simulink model "TB05_StageC_CLLC"  (R2025a)
settings: Solver=FixedStepDiscrete  StartTime=0  StopTime=TB.t_end  FixedStep=TB.dt  RelTol=1e-3
InitFcn:
  | % 모델과 같은 폴더의 초기화 스크립트를 실행해 P(설계 파라미터)와 TB(시험 조건)를 만든다.
  | run(fullfile(fileparts(get_param(bdroot, 'FileName')), 'TB05_init.m'));
values from neighbouring files (symbols this model uses):
  TB = struct()    [TB05_init.m]    (also in probe_TB05_solver.m = evalin('base', 'TB'); run_TB05.m = evalin('base', 'TB'))
libraries: fl_lib x35, nesl_utility x13
settings Model: Creator=hj000  LastModifiedBy=hj000
settings DataIOCC: SaveOutput=off  SignalLogging=off  SaveTime=off

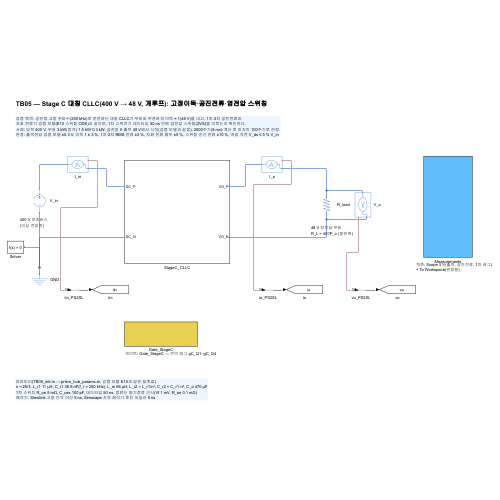
[thumbnail: Simulink's stored preview of the top-level diagram]
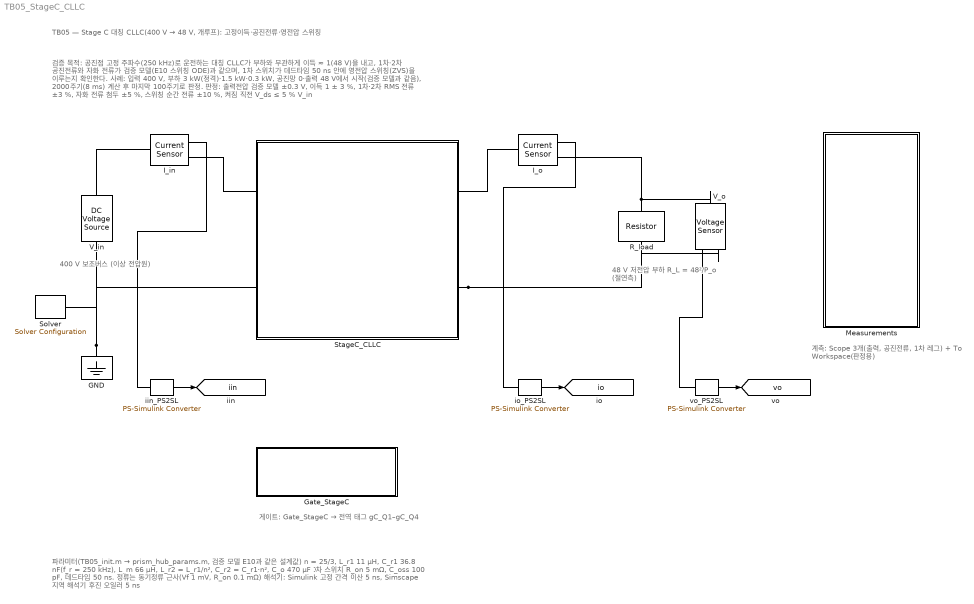
== system TB05_StageC_CLLC ==
  note: TB05 — Stage C 대칭 CLLC(400 V → 48 V, 개루프): 고정이득·공진전류·영전압 스위칭
  note: 검증 목적: 공진점 고정 주파수(250 kHz)로 운전하는 대칭 CLLC가 부하와 무관하게 이득 ≈ 1(48 V)을 내고, 1차·2차 공진전류와
      | 자화 전류가 검증 모델(E10 스위칭 ODE)과 같으며, 1차 스위치가 데드타임 50 ns 안에 영전압 스위칭(ZVS)을 이루는지 확인한다.
      | 사례: 입력 400 V, 부하 3 kW(정격)·1.5 kW·0.3 kW, 공진망 0·출력 48 V에서 시작(검증 모델과 같음), 2000주기(8 ms) 계산 후 마지막 100주기로 판정.
      | 판정: 출력전압 검증 모델 ±0.3 V, 이득 1 ± 3 %, 1차·2차 RMS 전류 ±3 %, 자화 전류 첨두 ±5 %, 스위칭 순간 전류 ±10 %, 켜짐 직전 V_ds ≤ 5 % V_in
  note: 400 V 보조버스
      | (이상 전압원)
  note: 48 V 저전압 부하
      | R_L = 48²/P_o (절연측)
  note: 게이트: Gate_StageC → 전역 태그 gC_Q1–gC_Q4
  note: 계측: Scope 3개(출력, 공진전류, 1차 레그)
      | + To Workspace(판정용)
  note: 파라미터(TB05_init.m → prism_hub_params.m, 검증 모델 E10과 같은 설계값)
      | n = 25/3, L_r1 11 µH, C_r1 36.8 nF(f_r = 250 kHz), L_m 66 µH, L_r2 = L_r1/n², C_r2 = C_r1·n², C_o 470 µF
      | 1차 스위치 R_on 5 mΩ, C_oss 100 pF, 데드타임 50 ns. 정류는 동기정류 근사(Vf 1 mV, R_on 0.1 mΩ)
      | 해석기: Simulink 고정 간격 이산 5 ns, Simscape 지역 해석기 후진 오일러 5 ns
  GND : fl_lib/Electrical/Electrical Elements/Electrical Reference
  Gate_StageC : Subsystem
  I_in : fl_lib/Electrical/Electrical Sensors/Current Sensor
  I_o : fl_lib/Electrical/Electrical Sensors/Current Sensor
  Measurements : Subsystem
  R_load : fl_lib/Electrical/Electrical Elements/Resistor  R=TB.RL Ohm  i_specify=off  i_priority=None  i=0 A  i_nominal_specify=off  i_nominal_value=1  i_nominal_unit=A  v_specify=off  v_priority=None  v=0 V  v_nominal_specify=off  v_nominal_value=1  v_nominal_unit=V
  Solver : nesl_utility/Solver Configuration  PhysicalDomain=network_engine_domain  SubClassName=solver  LeftPortType=input  RightPortType=generic  Tones=[]  Harmonics=[]  SimulateNoise=off  Profile=off  UseLocalSampling=off  EnableSwitchedLinearOptims=on  FrequencyDomain=off  UseCCode=off  RelTol=0.001  AbsTol=0.001  MinStep=1e-09  ToWorkspace=off  RevertToSquareIcSolve=off  NumHomotopyIterations=100  PhasorMode=off  PhasorModeNumHarmonics=1  ConsistencySolver=NEWTON_XTOL_AFTER_FTOL  IndexReductionMethod=DerivativeReplacement  DoDC=off  ResidualTolerance=1e-9  ConsistencyTolSource=GLOBAL  ConsistencyAbsTol=0.001  ConsistencyRelTol=0.001  ConsistencyTolFactor=0.001  UseLocalSolver=on  LocalSolverChoice=NE_BACKWARD_EULER_ADVANCER  ResolveIndetEquations=on  FunctionEvalNumThread=1  LocalSolverSampleTime=TB.dt  DoFixedCost=off  MaxNonlinIter=3  MaxModeIter=2  ComputeImpulses=off  ImpulseIterations=2  LinearAlgebra=auto  LinearAlgebraNumThread=0  EquationFormulation=NE_TIME_EF  DelaysMemoryBudget=1024  AutomaticFiltering=on  FilteringTimeConstant=0.001  PartitionStorageMethod=AS_NEEDED  PartitionMemoryBudget=1024  PartitionMethod=ROBUST  MultibodyUseLocalSolver=off  MultibodyLocalSolverChoice=ODE1  MultibodyLocalSolverSampleTime=0.001
  StageC_CLLC : Subsystem
  V_in : fl_lib/Electrical/Electrical Sources/DC Voltage Source  v0=TB.Vin V
  V_o : fl_lib/Electrical/Electrical Sensors/Voltage Sensor
  iin_PS2SL : nesl_utility/PS-Simulink Converter  PhysicalDomain=network_engine_domain  SubClassName=ps_output  LeftPortType=input  RightPortType=output  PseudoPeriodic=off  Frequencies=[]  VectorFormat=inherit  Unit=inherit  AffineConversion=off
  io_PS2SL : nesl_utility/PS-Simulink Converter  PhysicalDomain=network_engine_domain  SubClassName=ps_output  LeftPortType=input  RightPortType=output  PseudoPeriodic=off  Frequencies=[]  VectorFormat=inherit  Unit=inherit  AffineConversion=off
  vo_PS2SL : nesl_utility/PS-Simulink Converter  PhysicalDomain=network_engine_domain  SubClassName=ps_output  LeftPortType=input  RightPortType=output  PseudoPeriodic=off  Frequencies=[]  VectorFormat=inherit  Unit=inherit  AffineConversion=off
  tag scope: iin=global, io=global, vo=global
  wires:
  iin_PS2SL/1 -> [iin]
  io_PS2SL/1 -> [io]
  vo_PS2SL/1 -> [vo]
  connections:
  Solver/RConn1 -- V_in/RConn1 -- GND/LConn1 -- StageC_CLLC/LConn2
  V_in/LConn1 -- I_in/LConn1
  I_in/RConn2 -- StageC_CLLC/LConn1
  StageC_CLLC/RConn1 -- I_o/LConn1
  R_load/LConn1 -- I_o/RConn2 -- V_o/LConn1
  StageC_CLLC/RConn2 -- R_load/RConn1 -- V_o/RConn2
  I_in/RConn1 -- iin_PS2SL/LConn1
  I_o/RConn1 -- io_PS2SL/LConn1
  V_o/RConn1 -- vo_PS2SL/LConn1

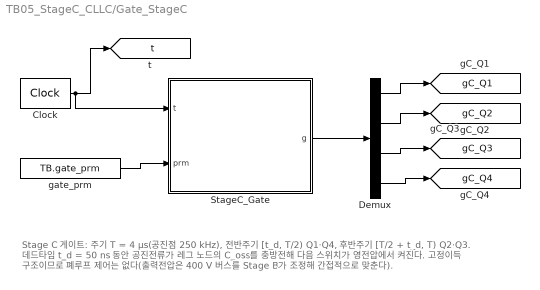
== system TB05_StageC_CLLC/Gate_StageC ==
  note: Stage C 게이트: 주기 T = 4 µs(공진점 250 kHz), 전반주기 [t_d, T/2) Q1·Q4, 후반주기 [T/2 + t_d, T) Q2·Q3.
      | 데드타임 t_d = 50 ns 동안 공진전류가 레그 노드의 C_oss를 충방전해 다음 스위치가 영전압에서 켜진다.
      | 고정이득 구조이므로 폐루프 제어는 없다(출력전압은 400 V 버스를 Stage B가 조정해 간접적으로 맞춘다).
  Clock : DigitalClock  SampleTime=TB.dt
  Demux : Demux
  StageC_Gate : MATLAB Function  TreatAsAtomicUnit=on
  gate_prm : Constant  Value=TB.gate_prm
  tag scope: gC_Q1=global, gC_Q2=global, gC_Q3=global, gC_Q4=global, t=global
  wires:
  Clock/1 -> [t], StageC_Gate/1(t)
  gate_prm/1 -> StageC_Gate/2(prm)
  StageC_Gate/1(g) -> Demux/1
  Demux/1 -> [gC_Q1]
  Demux/2 -> [gC_Q2]
  Demux/3 -> [gC_Q3]
  Demux/4 -> [gC_Q4]

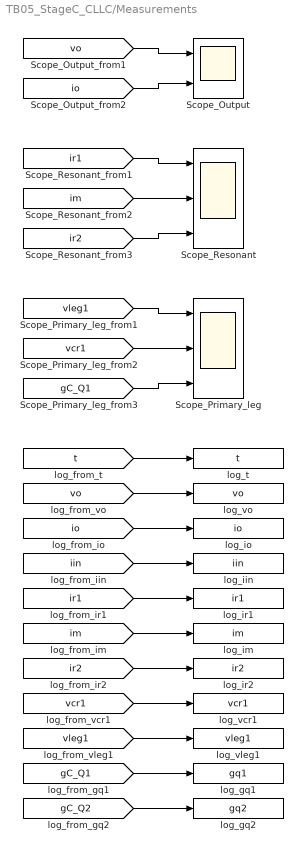
== system TB05_StageC_CLLC/Measurements ==
  Scope_Output : Scope  NumInputPorts=2
      settings: Title=Scope Output
  Scope_Primary_leg : Scope  NumInputPorts=3
      settings: Title=Scope Primary leg
  Scope_Resonant : Scope  NumInputPorts=3
      settings: Title=Scope Resonant
  log_gq1 : ToWorkspace  VariableName=gq1  SampleTime=-1
  log_gq2 : ToWorkspace  VariableName=gq2  SampleTime=-1
  log_iin : ToWorkspace  VariableName=iin  SampleTime=-1
  log_im : ToWorkspace  VariableName=im  SampleTime=-1
  log_io : ToWorkspace  VariableName=io  SampleTime=-1
  log_ir1 : ToWorkspace  VariableName=ir1  SampleTime=-1
  log_ir2 : ToWorkspace  VariableName=ir2  SampleTime=-1
  log_t : ToWorkspace  VariableName=t  SampleTime=-1
  log_vcr1 : ToWorkspace  VariableName=vcr1  SampleTime=-1
  log_vleg1 : ToWorkspace  VariableName=vleg1  SampleTime=-1
  log_vo : ToWorkspace  VariableName=vo  SampleTime=-1
  wires:
  [vo] -> Scope_Output/1
  [io] -> Scope_Output/2
  [ir1] -> Scope_Resonant/1
  [im] -> Scope_Resonant/2
  [ir2] -> Scope_Resonant/3
  [vleg1] -> Scope_Primary_leg/1
  [vcr1] -> Scope_Primary_leg/2
  [gC_Q1] -> Scope_Primary_leg/3
  [t] -> log_t/1
  [vo] -> log_vo/1
  [io] -> log_io/1
  [iin] -> log_iin/1
  [ir1] -> log_ir1/1
  [im] -> log_im/1
  [ir2] -> log_ir2/1
  [vcr1] -> log_vcr1/1
  [vleg1] -> log_vleg1/1
  [gC_Q1] -> log_gq1/1
  [gC_Q2] -> log_gq2/1

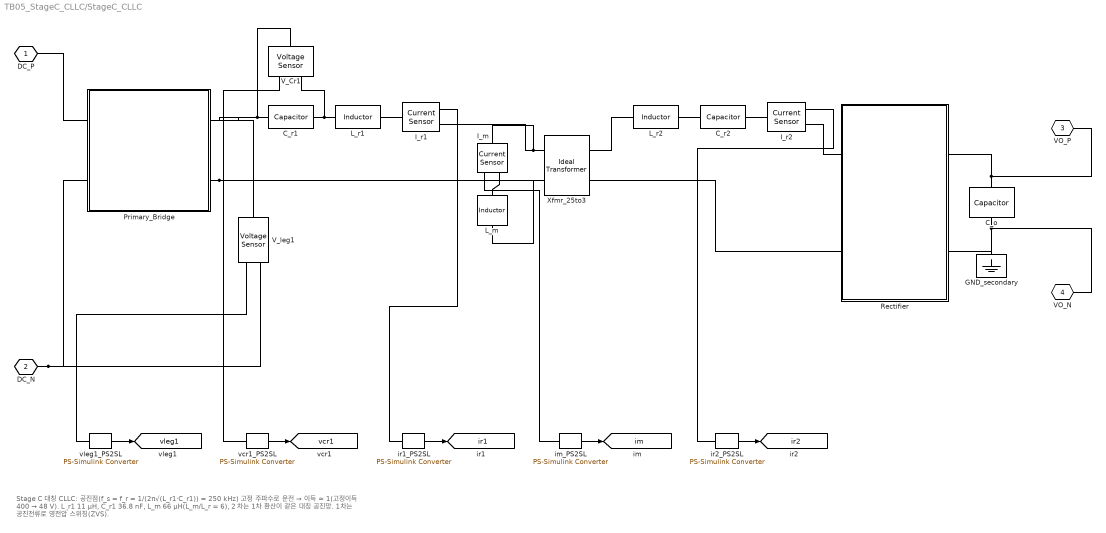
== system TB05_StageC_CLLC/StageC_CLLC ==
  note: Stage C 대칭 CLLC: 공진점(f_s = f_r = 1/(2π√(L_r1·C_r1)) = 250 kHz) 고정 주파수로 운전 → 이득 ≈ 1(고정이득 400 → 48 V).
      | L_r1 11 µH, C_r1 36.8 nF, L_m 66 µH(L_m/L_r = 6), 2차는 1차 환산이 같은 대칭 공진망. 1차는 공진전류로 영전압 스위칭(ZVS).
  C_o : fl_lib/Electrical/Electrical Elements/Capacitor  c=TB.C.Co F  r=1e-6 Ohm  g=0 1/Ohm  i_specify=off  i_priority=None  i=0 A  i_nominal_specify=off  i_nominal_value=1  i_nominal_unit=A  v_specify=off  v_priority=None  v=0 V  v_nominal_specify=off  v_nominal_value=1  v_nominal_unit=V  vc_specify=on  vc_priority=High  vc=TB.vo0 V  vc_nominal_specify=off  vc_nominal_value=1  vc_nominal_unit=V
  C_r1 : fl_lib/Electrical/Electrical Elements/Capacitor  c=TB.C.Cr1 F  r=1e-6 Ohm  g=0 1/Ohm  i_specify=off  i_priority=None  i=0 A  i_nominal_specify=off  i_nominal_value=1  i_nominal_unit=A  v_specify=off  v_priority=None  v=0 V  v_nominal_specify=off  v_nominal_value=1  v_nominal_unit=V  vc_specify=on  vc_priority=High  vc=0 V  vc_nominal_specify=off  vc_nominal_value=1  vc_nominal_unit=V
  C_r2 : fl_lib/Electrical/Electrical Elements/Capacitor  c=TB.C.Cr2 F  r=1e-6 Ohm  g=0 1/Ohm  i_specify=off  i_priority=None  i=0 A  i_nominal_specify=off  i_nominal_value=1  i_nominal_unit=A  v_specify=off  v_priority=None  v=0 V  v_nominal_specify=off  v_nominal_value=1  v_nominal_unit=V  vc_specify=on  vc_priority=High  vc=0 V  vc_nominal_specify=off  vc_nominal_value=1  vc_nominal_unit=V
  GND_secondary : fl_lib/Electrical/Electrical Elements/Electrical Reference
  I_m : fl_lib/Electrical/Electrical Sensors/Current Sensor
  I_r1 : fl_lib/Electrical/Electrical Sensors/Current Sensor
  I_r2 : fl_lib/Electrical/Electrical Sensors/Current Sensor
  L_m : fl_lib/Electrical/Electrical Elements/Inductor  l=TB.C.Lm H  r=0 Ohm  g=1e-9 1/Ohm  i_specify=off  i_priority=None  i=0 A  i_nominal_specify=off  i_nominal_value=1  i_nominal_unit=A  v_specify=off  v_priority=None  v=0 V  v_nominal_specify=off  v_nominal_value=1  v_nominal_unit=V  i_L_specify=on  i_L_priority=High  i_L=0 A  i_L_nominal_specify=off  i_L_nominal_value=1  i_L_nominal_unit=A
  L_r1 : fl_lib/Electrical/Electrical Elements/Inductor  l=TB.C.Lr1 H  r=0 Ohm  g=1e-9 1/Ohm  i_specify=off  i_priority=None  i=0 A  i_nominal_specify=off  i_nominal_value=1  i_nominal_unit=A  v_specify=off  v_priority=None  v=0 V  v_nominal_specify=off  v_nominal_value=1  v_nominal_unit=V  i_L_specify=on  i_L_priority=High  i_L=0 A  i_L_nominal_specify=off  i_L_nominal_value=1  i_L_nominal_unit=A
  L_r2 : fl_lib/Electrical/Electrical Elements/Inductor  l=TB.C.Lr2 H  r=0 Ohm  g=1e-9 1/Ohm  i_specify=off  i_priority=None  i=0 A  i_nominal_specify=off  i_nominal_value=1  i_nominal_unit=A  v_specify=off  v_priority=None  v=0 V  v_nominal_specify=off  v_nominal_value=1  v_nominal_unit=V  i_L_specify=on  i_L_priority=High  i_L=0 A  i_L_nominal_specify=off  i_L_nominal_value=1  i_L_nominal_unit=A
  Primary_Bridge : Subsystem
  Rectifier : Subsystem
  V_Cr1 : fl_lib/Electrical/Electrical Sensors/Voltage Sensor
  V_leg1 : fl_lib/Electrical/Electrical Sensors/Voltage Sensor
  Xfmr_25to3 : fl_lib/Electrical/Electrical Elements/Ideal Transformer  n=TB.C.n  i1_specify=off  i1_priority=None  i1=0 A  i1_nominal_specify=off  i1_nominal_value=1  i1_nominal_unit=A  v1_specify=off  v1_priority=None  v1=0 V  v1_nominal_specify=off  v1_nominal_value=1  v1_nominal_unit=V  i2_specify=off  i2_priority=None  i2=0 A  i2_nominal_specify=off  i2_nominal_value=1  i2_nominal_unit=A  v2_specify=off  v2_priority=None  v2=0 V  v2_nominal_specify=off  v2_nominal_value=1  v2_nominal_unit=V
  im_PS2SL : nesl_utility/PS-Simulink Converter  PhysicalDomain=network_engine_domain  SubClassName=ps_output  LeftPortType=input  RightPortType=output  PseudoPeriodic=off  Frequencies=[]  VectorFormat=inherit  Unit=inherit  AffineConversion=off
  ir1_PS2SL : nesl_utility/PS-Simulink Converter  PhysicalDomain=network_engine_domain  SubClassName=ps_output  LeftPortType=input  RightPortType=output  PseudoPeriodic=off  Frequencies=[]  VectorFormat=inherit  Unit=inherit  AffineConversion=off
  ir2_PS2SL : nesl_utility/PS-Simulink Converter  PhysicalDomain=network_engine_domain  SubClassName=ps_output  LeftPortType=input  RightPortType=output  PseudoPeriodic=off  Frequencies=[]  VectorFormat=inherit  Unit=inherit  AffineConversion=off
  vcr1_PS2SL : nesl_utility/PS-Simulink Converter  PhysicalDomain=network_engine_domain  SubClassName=ps_output  LeftPortType=input  RightPortType=output  PseudoPeriodic=off  Frequencies=[]  VectorFormat=inherit  Unit=inherit  AffineConversion=off
  vleg1_PS2SL : nesl_utility/PS-Simulink Converter  PhysicalDomain=network_engine_domain  SubClassName=ps_output  LeftPortType=input  RightPortType=output  PseudoPeriodic=off  Frequencies=[]  VectorFormat=inherit  Unit=inherit  AffineConversion=off
  DC_P : PMIOPort  Side=Left
  DC_N : PMIOPort  Port=2  Side=Left
  VO_P : PMIOPort  Port=3  Side=Right
  VO_N : PMIOPort  Port=4  Side=Right
  tag scope: im=global, ir1=global, ir2=global, vcr1=global, vleg1=global
  wires:
  ir1_PS2SL/1 -> [ir1]
  im_PS2SL/1 -> [im]
  ir2_PS2SL/1 -> [ir2]
  vcr1_PS2SL/1 -> [vcr1]
  vleg1_PS2SL/1 -> [vleg1]
  connections:
  Primary_Bridge/LConn1 -- DC_P/RConn1
  DC_N/RConn1 -- Primary_Bridge/LConn2 -- V_leg1/RConn2
  C_r1/LConn1 -- Primary_Bridge/RConn1 -- V_leg1/LConn1 -- V_Cr1/LConn1
  L_r1/LConn1 -- C_r1/RConn1 -- V_Cr1/RConn2
  L_r1/RConn1 -- I_r1/LConn1
  Xfmr_25to3/LConn1 -- I_r1/RConn2 -- I_m/LConn1
  Primary_Bridge/RConn2 -- Xfmr_25to3/LConn2 -- L_m/RConn1
  I_m/RConn2 -- L_m/LConn1
  Xfmr_25to3/RConn1 -- L_r2/LConn1
  L_r2/RConn1 -- C_r2/LConn1
  C_r2/RConn1 -- I_r2/LConn1
  I_r2/RConn2 -- Rectifier/LConn1
  Xfmr_25to3/RConn2 -- Rectifier/LConn2
  C_o/LConn1 -- Rectifier/RConn1 -- VO_P/RConn1
  Rectifier/RConn2 -- VO_N/RConn1 -- C_o/RConn1 -- GND_secondary/LConn1
  I_r1/RConn1 -- ir1_PS2SL/LConn1
  I_m/RConn1 -- im_PS2SL/LConn1
  I_r2/RConn1 -- ir2_PS2SL/LConn1
  V_Cr1/RConn1 -- vcr1_PS2SL/LConn1
  V_leg1/RConn1 -- vleg1_PS2SL/LConn1

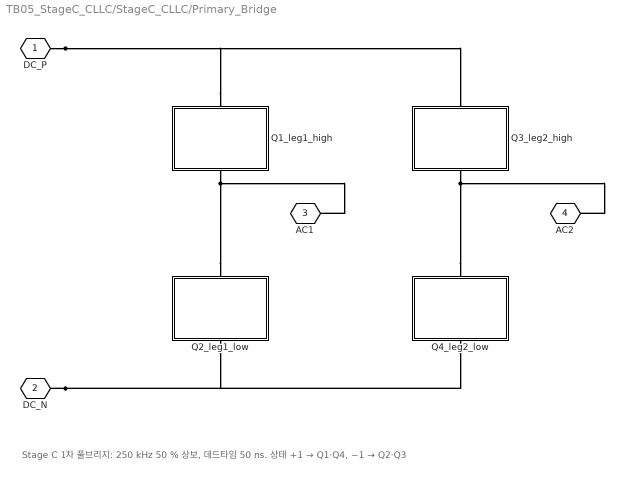
== system TB05_StageC_CLLC/StageC_CLLC/Primary_Bridge ==
  note: Stage C 1차 풀브리지: 250 kHz 50 % 상보, 데드타임 50 ns. 상태 +1 → Q1·Q4, −1 → Q2·Q3
  Q1_leg1_high : Subsystem  mask(PRISM-Hub switch cell){Ron=TB.C.Ron, Goff=TB.C.Goff, Vf=TB.C.Vf, Rd=TB.C.Rd, Goffd=TB.C.Goffd, Coss=TB.C.Coss}
      mask prompts: Ron "도통 저항 R_on [Ohm]"; Goff "차단 컨덕턴스 G_off [S]"; Vf "다이오드 순방향 전압 Vf [V]"; Rd "다이오드 도통 저항 R_d [Ohm]"; Goffd "다이오드 차단 컨덕턴스 [S]"; Coss "출력용량 C_oss [F]"
      mask help: 전력 반도체 스위치 셀 Q1_leg1_high. 게이트 태그 gC_Q1.
      settings: AttributesFormatString=gate: gC_Q1
      mask Display:
      | plot([0.50 0.50 ],[0.95 0.65 ],[0.50 0.74 ],[0.65 0.35 ],[0.50 0.50 ],[0.35 0.05 ]);
      | plot([0.50 0.20 0.20 ],[0.80 0.80 0.58 ],[0.20 0.20 0.50 ],[0.42 0.20 0.20 ]);
      | plot([0.20 0.10 0.30 0.20 ],[0.58 0.42 0.42 0.58 ],[0.10 0.30 ],[0.58 0.58 ]);
      | port_label('LConn',1,'D');
      | port_label('RConn',1,'S');
  Q2_leg1_low : Subsystem  mask(PRISM-Hub switch cell){Ron=TB.C.Ron, Goff=TB.C.Goff, Vf=TB.C.Vf, Rd=TB.C.Rd, Goffd=TB.C.Goffd, Coss=TB.C.Coss}
      mask prompts: Ron "도통 저항 R_on [Ohm]"; Goff "차단 컨덕턴스 G_off [S]"; Vf "다이오드 순방향 전압 Vf [V]"; Rd "다이오드 도통 저항 R_d [Ohm]"; Goffd "다이오드 차단 컨덕턴스 [S]"; Coss "출력용량 C_oss [F]"
      mask help: 전력 반도체 스위치 셀 Q2_leg1_low. 게이트 태그 gC_Q2.
      settings: AttributesFormatString=gate: gC_Q2
      mask Display:
      | plot([0.50 0.50 ],[0.95 0.65 ],[0.50 0.74 ],[0.65 0.35 ],[0.50 0.50 ],[0.35 0.05 ]);
      | plot([0.50 0.20 0.20 ],[0.80 0.80 0.58 ],[0.20 0.20 0.50 ],[0.42 0.20 0.20 ]);
      | plot([0.20 0.10 0.30 0.20 ],[0.58 0.42 0.42 0.58 ],[0.10 0.30 ],[0.58 0.58 ]);
      | port_label('LConn',1,'D');
      | port_label('RConn',1,'S');
  Q3_leg2_high : Subsystem  mask(PRISM-Hub switch cell){Ron=TB.C.Ron, Goff=TB.C.Goff, Vf=TB.C.Vf, Rd=TB.C.Rd, Goffd=TB.C.Goffd, Coss=TB.C.Coss}
      mask prompts: Ron "도통 저항 R_on [Ohm]"; Goff "차단 컨덕턴스 G_off [S]"; Vf "다이오드 순방향 전압 Vf [V]"; Rd "다이오드 도통 저항 R_d [Ohm]"; Goffd "다이오드 차단 컨덕턴스 [S]"; Coss "출력용량 C_oss [F]"
      mask help: 전력 반도체 스위치 셀 Q3_leg2_high. 게이트 태그 gC_Q3.
      settings: AttributesFormatString=gate: gC_Q3
      mask Display:
      | plot([0.50 0.50 ],[0.95 0.65 ],[0.50 0.74 ],[0.65 0.35 ],[0.50 0.50 ],[0.35 0.05 ]);
      | plot([0.50 0.20 0.20 ],[0.80 0.80 0.58 ],[0.20 0.20 0.50 ],[0.42 0.20 0.20 ]);
      | plot([0.20 0.10 0.30 0.20 ],[0.58 0.42 0.42 0.58 ],[0.10 0.30 ],[0.58 0.58 ]);
      | port_label('LConn',1,'D');
      | port_label('RConn',1,'S');
  Q4_leg2_low : Subsystem  mask(PRISM-Hub switch cell){Ron=TB.C.Ron, Goff=TB.C.Goff, Vf=TB.C.Vf, Rd=TB.C.Rd, Goffd=TB.C.Goffd, Coss=TB.C.Coss}
      mask prompts: Ron "도통 저항 R_on [Ohm]"; Goff "차단 컨덕턴스 G_off [S]"; Vf "다이오드 순방향 전압 Vf [V]"; Rd "다이오드 도통 저항 R_d [Ohm]"; Goffd "다이오드 차단 컨덕턴스 [S]"; Coss "출력용량 C_oss [F]"
      mask help: 전력 반도체 스위치 셀 Q4_leg2_low. 게이트 태그 gC_Q4.
      settings: AttributesFormatString=gate: gC_Q4
      mask Display:
      | plot([0.50 0.50 ],[0.95 0.65 ],[0.50 0.74 ],[0.65 0.35 ],[0.50 0.50 ],[0.35 0.05 ]);
      | plot([0.50 0.20 0.20 ],[0.80 0.80 0.58 ],[0.20 0.20 0.50 ],[0.42 0.20 0.20 ]);
      | plot([0.20 0.10 0.30 0.20 ],[0.58 0.42 0.42 0.58 ],[0.10 0.30 ],[0.58 0.58 ]);
      | port_label('LConn',1,'D');
      | port_label('RConn',1,'S');
  DC_P : PMIOPort  Side=Left
  DC_N : PMIOPort  Port=2  Side=Left
  AC1 : PMIOPort  Port=3  Side=Right
  AC2 : PMIOPort  Port=4  Side=Right
  connections:
  Q1_leg1_high/LConn1 -- DC_P/RConn1 -- Q3_leg2_high/LConn1
  Q2_leg1_low/LConn1 -- Q1_leg1_high/RConn1 -- AC1/RConn1
  Q4_leg2_low/LConn1 -- Q3_leg2_high/RConn1 -- AC2/RConn1
  DC_N/RConn1 -- Q2_leg1_low/RConn1 -- Q4_leg2_low/RConn1

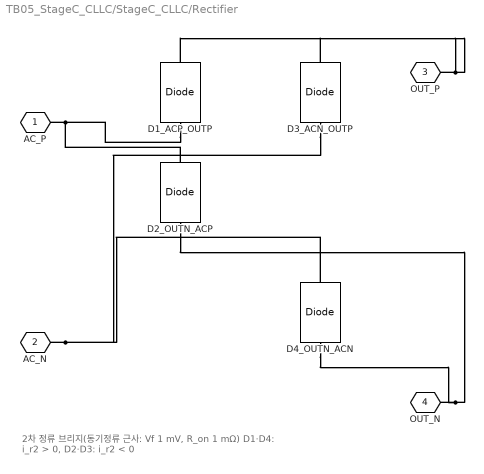
== system TB05_StageC_CLLC/StageC_CLLC/Rectifier ==
  note: 2차 정류 브리지(동기정류 근사: Vf 1 mV, R_on 1 mΩ)
      | D1·D4: i_r2 > 0, D2·D3: i_r2 < 0
  D1_ACP_OUTP : fl_lib/Electrical/Electrical Elements/Diode  Vf=TB.C.Vf_rect V  Ron=TB.C.Ron_rect Ohm  Goff=1e-8 1/Ohm  i_specify=off  i_priority=None  i=0 A  i_nominal_specify=off  i_nominal_value=1  i_nominal_unit=A  v_specify=off  v_priority=None  v=0 V  v_nominal_specify=off  v_nominal_value=1  v_nominal_unit=V
  D2_OUTN_ACP : fl_lib/Electrical/Electrical Elements/Diode  Vf=TB.C.Vf_rect V  Ron=TB.C.Ron_rect Ohm  Goff=1e-8 1/Ohm  i_specify=off  i_priority=None  i=0 A  i_nominal_specify=off  i_nominal_value=1  i_nominal_unit=A  v_specify=off  v_priority=None  v=0 V  v_nominal_specify=off  v_nominal_value=1  v_nominal_unit=V
  D3_ACN_OUTP : fl_lib/Electrical/Electrical Elements/Diode  Vf=TB.C.Vf_rect V  Ron=TB.C.Ron_rect Ohm  Goff=1e-8 1/Ohm  i_specify=off  i_priority=None  i=0 A  i_nominal_specify=off  i_nominal_value=1  i_nominal_unit=A  v_specify=off  v_priority=None  v=0 V  v_nominal_specify=off  v_nominal_value=1  v_nominal_unit=V
  D4_OUTN_ACN : fl_lib/Electrical/Electrical Elements/Diode  Vf=TB.C.Vf_rect V  Ron=TB.C.Ron_rect Ohm  Goff=1e-8 1/Ohm  i_specify=off  i_priority=None  i=0 A  i_nominal_specify=off  i_nominal_value=1  i_nominal_unit=A  v_specify=off  v_priority=None  v=0 V  v_nominal_specify=off  v_nominal_value=1  v_nominal_unit=V
  AC_P : PMIOPort  Side=Left
  AC_N : PMIOPort  Port=2  Side=Left
  OUT_P : PMIOPort  Port=3  Side=Right
  OUT_N : PMIOPort  Port=4  Side=Right
  connections:
  AC_P/RConn1 -- D1_ACP_OUTP/LConn1 -- D2_OUTN_ACP/RConn1
  OUT_P/RConn1 -- D1_ACP_OUTP/RConn1 -- D3_ACN_OUTP/RConn1
  OUT_N/RConn1 -- D2_OUTN_ACP/LConn1 -- D4_OUTN_ACN/LConn1
  AC_N/RConn1 -- D3_ACN_OUTP/LConn1 -- D4_OUTN_ACN/RConn1

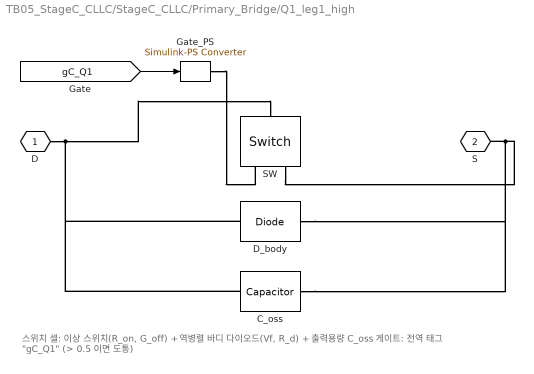
== system TB05_StageC_CLLC/StageC_CLLC/Primary_Bridge/Q1_leg1_high ==
  note: 스위치 셀: 이상 스위치(R_on, G_off) + 역병렬 바디 다이오드(Vf, R_d) + 출력용량 C_oss
      | 게이트: 전역 태그 "gC_Q1" (> 0.5 이면 도통)
  C_oss : fl_lib/Electrical/Electrical Elements/Capacitor  c=Coss F  r=1e-6 Ohm  g=0 1/Ohm  i_specify=off  i_priority=None  i=0 A  i_nominal_specify=off  i_nominal_value=1  i_nominal_unit=A  v_specify=off  v_priority=None  v=0 V  v_nominal_specify=off  v_nominal_value=1  v_nominal_unit=V  vc_specify=off  vc_priority=High  vc=0 V  vc_nominal_specify=off  vc_nominal_value=1  vc_nominal_unit=V
  D_body : fl_lib/Electrical/Electrical Elements/Diode  Vf=Vf V  Ron=Rd Ohm  Goff=Goffd 1/Ohm  i_specify=off  i_priority=None  i=0 A  i_nominal_specify=off  i_nominal_value=1  i_nominal_unit=A  v_specify=off  v_priority=None  v=0 V  v_nominal_specify=off  v_nominal_value=1  v_nominal_unit=V
  Gate_PS : nesl_utility/Simulink-PS Converter  PhysicalDomain=network_engine_domain  SubClassName=ps_input  LeftPortType=input  RightPortType=output  PseudoPeriodic=off  Frequencies=[]  NoiseDistribution=none  NoiseParameters=[]  Unit=1  AffineConversion=off  FilteringAndDerivatives=zero  SimscapeFilterOrder=1  InputFilterTimeConstant=0.001  UdotUserProvided=0
  SW : fl_lib/Electrical/Electrical Elements/Switch  R_closed=Ron Ohm  G_open=Goff 1/Ohm  Threshold=0.5  i_specify=off  i_priority=None  i=0 A  i_nominal_specify=off  i_nominal_value=1  i_nominal_unit=A  v_specify=off  v_priority=None  v=0 V  v_nominal_specify=off  v_nominal_value=1  v_nominal_unit=V
  D : PMIOPort  Side=Left
  S : PMIOPort  Port=2  Side=Right
  wires:
  [gC_Q1] -> Gate_PS/1
  connections:
  Gate_PS/RConn1 -- SW/RConn1
  SW/LConn1 -- D/RConn1 -- D_body/RConn1 -- C_oss/LConn1
  SW/RConn2 -- D_body/LConn1 -- S/RConn1 -- C_oss/RConn1

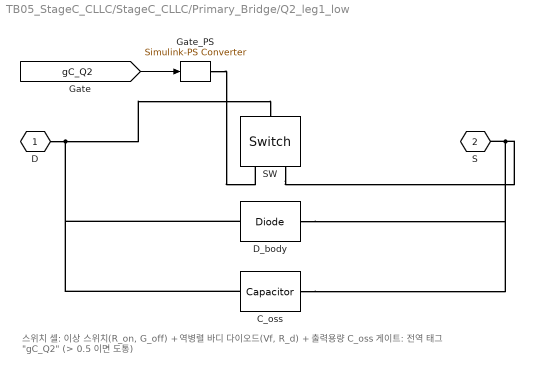
== system TB05_StageC_CLLC/StageC_CLLC/Primary_Bridge/Q2_leg1_low ==
  note: 스위치 셀: 이상 스위치(R_on, G_off) + 역병렬 바디 다이오드(Vf, R_d) + 출력용량 C_oss
      | 게이트: 전역 태그 "gC_Q2" (> 0.5 이면 도통)
  C_oss : fl_lib/Electrical/Electrical Elements/Capacitor  c=Coss F  r=1e-6 Ohm  g=0 1/Ohm  i_specify=off  i_priority=None  i=0 A  i_nominal_specify=off  i_nominal_value=1  i_nominal_unit=A  v_specify=off  v_priority=None  v=0 V  v_nominal_specify=off  v_nominal_value=1  v_nominal_unit=V  vc_specify=off  vc_priority=High  vc=0 V  vc_nominal_specify=off  vc_nominal_value=1  vc_nominal_unit=V
  D_body : fl_lib/Electrical/Electrical Elements/Diode  Vf=Vf V  Ron=Rd Ohm  Goff=Goffd 1/Ohm  i_specify=off  i_priority=None  i=0 A  i_nominal_specify=off  i_nominal_value=1  i_nominal_unit=A  v_specify=off  v_priority=None  v=0 V  v_nominal_specify=off  v_nominal_value=1  v_nominal_unit=V
  Gate_PS : nesl_utility/Simulink-PS Converter  PhysicalDomain=network_engine_domain  SubClassName=ps_input  LeftPortType=input  RightPortType=output  PseudoPeriodic=off  Frequencies=[]  NoiseDistribution=none  NoiseParameters=[]  Unit=1  AffineConversion=off  FilteringAndDerivatives=zero  SimscapeFilterOrder=1  InputFilterTimeConstant=0.001  UdotUserProvided=0
  SW : fl_lib/Electrical/Electrical Elements/Switch  R_closed=Ron Ohm  G_open=Goff 1/Ohm  Threshold=0.5  i_specify=off  i_priority=None  i=0 A  i_nominal_specify=off  i_nominal_value=1  i_nominal_unit=A  v_specify=off  v_priority=None  v=0 V  v_nominal_specify=off  v_nominal_value=1  v_nominal_unit=V
  D : PMIOPort  Side=Left
  S : PMIOPort  Port=2  Side=Right
  wires:
  [gC_Q2] -> Gate_PS/1
  connections:
  Gate_PS/RConn1 -- SW/RConn1
  SW/LConn1 -- D/RConn1 -- D_body/RConn1 -- C_oss/LConn1
  SW/RConn2 -- D_body/LConn1 -- S/RConn1 -- C_oss/RConn1

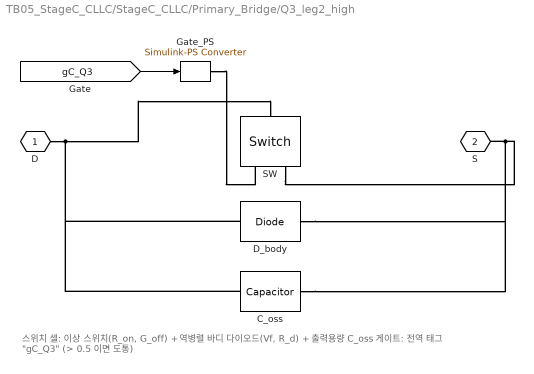
== system TB05_StageC_CLLC/StageC_CLLC/Primary_Bridge/Q3_leg2_high ==
  note: 스위치 셀: 이상 스위치(R_on, G_off) + 역병렬 바디 다이오드(Vf, R_d) + 출력용량 C_oss
      | 게이트: 전역 태그 "gC_Q3" (> 0.5 이면 도통)
  C_oss : fl_lib/Electrical/Electrical Elements/Capacitor  c=Coss F  r=1e-6 Ohm  g=0 1/Ohm  i_specify=off  i_priority=None  i=0 A  i_nominal_specify=off  i_nominal_value=1  i_nominal_unit=A  v_specify=off  v_priority=None  v=0 V  v_nominal_specify=off  v_nominal_value=1  v_nominal_unit=V  vc_specify=off  vc_priority=High  vc=0 V  vc_nominal_specify=off  vc_nominal_value=1  vc_nominal_unit=V
  D_body : fl_lib/Electrical/Electrical Elements/Diode  Vf=Vf V  Ron=Rd Ohm  Goff=Goffd 1/Ohm  i_specify=off  i_priority=None  i=0 A  i_nominal_specify=off  i_nominal_value=1  i_nominal_unit=A  v_specify=off  v_priority=None  v=0 V  v_nominal_specify=off  v_nominal_value=1  v_nominal_unit=V
  Gate_PS : nesl_utility/Simulink-PS Converter  PhysicalDomain=network_engine_domain  SubClassName=ps_input  LeftPortType=input  RightPortType=output  PseudoPeriodic=off  Frequencies=[]  NoiseDistribution=none  NoiseParameters=[]  Unit=1  AffineConversion=off  FilteringAndDerivatives=zero  SimscapeFilterOrder=1  InputFilterTimeConstant=0.001  UdotUserProvided=0
  SW : fl_lib/Electrical/Electrical Elements/Switch  R_closed=Ron Ohm  G_open=Goff 1/Ohm  Threshold=0.5  i_specify=off  i_priority=None  i=0 A  i_nominal_specify=off  i_nominal_value=1  i_nominal_unit=A  v_specify=off  v_priority=None  v=0 V  v_nominal_specify=off  v_nominal_value=1  v_nominal_unit=V
  D : PMIOPort  Side=Left
  S : PMIOPort  Port=2  Side=Right
  wires:
  [gC_Q3] -> Gate_PS/1
  connections:
  Gate_PS/RConn1 -- SW/RConn1
  SW/LConn1 -- D/RConn1 -- D_body/RConn1 -- C_oss/LConn1
  SW/RConn2 -- D_body/LConn1 -- S/RConn1 -- C_oss/RConn1

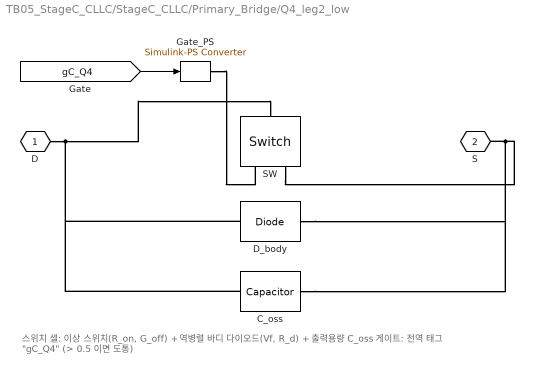
== system TB05_StageC_CLLC/StageC_CLLC/Primary_Bridge/Q4_leg2_low ==
  note: 스위치 셀: 이상 스위치(R_on, G_off) + 역병렬 바디 다이오드(Vf, R_d) + 출력용량 C_oss
      | 게이트: 전역 태그 "gC_Q4" (> 0.5 이면 도통)
  C_oss : fl_lib/Electrical/Electrical Elements/Capacitor  c=Coss F  r=1e-6 Ohm  g=0 1/Ohm  i_specify=off  i_priority=None  i=0 A  i_nominal_specify=off  i_nominal_value=1  i_nominal_unit=A  v_specify=off  v_priority=None  v=0 V  v_nominal_specify=off  v_nominal_value=1  v_nominal_unit=V  vc_specify=off  vc_priority=High  vc=0 V  vc_nominal_specify=off  vc_nominal_value=1  vc_nominal_unit=V
  D_body : fl_lib/Electrical/Electrical Elements/Diode  Vf=Vf V  Ron=Rd Ohm  Goff=Goffd 1/Ohm  i_specify=off  i_priority=None  i=0 A  i_nominal_specify=off  i_nominal_value=1  i_nominal_unit=A  v_specify=off  v_priority=None  v=0 V  v_nominal_specify=off  v_nominal_value=1  v_nominal_unit=V
  Gate_PS : nesl_utility/Simulink-PS Converter  PhysicalDomain=network_engine_domain  SubClassName=ps_input  LeftPortType=input  RightPortType=output  PseudoPeriodic=off  Frequencies=[]  NoiseDistribution=none  NoiseParameters=[]  Unit=1  AffineConversion=off  FilteringAndDerivatives=zero  SimscapeFilterOrder=1  InputFilterTimeConstant=0.001  UdotUserProvided=0
  SW : fl_lib/Electrical/Electrical Elements/Switch  R_closed=Ron Ohm  G_open=Goff 1/Ohm  Threshold=0.5  i_specify=off  i_priority=None  i=0 A  i_nominal_specify=off  i_nominal_value=1  i_nominal_unit=A  v_specify=off  v_priority=None  v=0 V  v_nominal_specify=off  v_nominal_value=1  v_nominal_unit=V
  D : PMIOPort  Side=Left
  S : PMIOPort  Port=2  Side=Right
  wires:
  [gC_Q4] -> Gate_PS/1
  connections:
  Gate_PS/RConn1 -- SW/RConn1
  SW/LConn1 -- D/RConn1 -- D_body/RConn1 -- C_oss/LConn1
  SW/RConn2 -- D_body/LConn1 -- S/RConn1 -- C_oss/RConn1

== matlab function TB05_StageC_CLLC/Gate_StageC/StageC_Gate ==
  data: t input; g output; prm input
function g = prism_gate_stageC(t, prm)
%#codegen
%PRISM_GATE_STAGEC  Stage C(대칭 CLLC) 1차 풀브리지 게이트: 공진점 고정 주파수, 50 % 상보 구형파 + 데드타임.
%
%   전반주기 [t_d, T/2)      : Q1(레그 1 상측)·Q4(레그 2 하측) 도통 → 1차 브리지 출력 +V_in
%   후반주기 [T/2 + t_d, T)  : Q2(레그 1 하측)·Q3(레그 2 상측) 도통 → −V_in
%   데드타임 동안 공진전류가 레그 노드의 출력용량을 충방전해 다음 소자가 영전압에서 켜진다(ZVS).
%   Stage C는 400 V 버스를 고정이득(권선비 25/3)으로 48 V로 바꾸므로 폐루프 제어 없이 이 타이밍만 쓴다.
%
%   입력  t    시각 [s] (Digital Clock, 간격 dt)
%         prm  [dt T t_d enable]  (T = 1/250 kHz, t_d = 50 ns)
%   출력  g    [Q1 Q2 Q3 Q4] (1 = 켬)

dt = prm(1); T = prm(2); td = prm(3);
g = zeros(4, 1);
if prm(4) > 0.5
    t0 = round(t/dt)*dt;                     % 적분 간격 격자 시각
    tau = mod(t0 + 1e-3*dt, T);              % 주기 안 위치(작은 치우침으로 경계 반올림 오차 흡수)
    on1 = (tau >= td) && (tau < T/2);
    on2 = (tau >= T/2 + td) && (tau < T);
    g = double([on1; on2; on2; on1]);
end
end
